simulink model "NBMS_SoC"  (R2026b)
settings: Solver=FixedStepDiscrete  StopTime=25  FixedStep=0.1
undefined symbols (not defined in the file): BMS_BattSoCDerate_E, BMS_BattTempDerate_E, BMS_MODE_E, CAL_15_SOC_WRN_RVL_THRSH, CAL_15_SOC_WRN_THRSH, CAL_DCHRG_END_THRSH, CAL_DOD, CAL_DOD_MAX_THRSH, CAL_DOD_MIN_THRSH, CAL_ENABLE_SOC_WARN_15, CAL_ENABLE_SOC_WARN_20, CAL_GOLDEN_CHARGE, CAL_GOLDEN_DC, CAL_LOW_SOC_RVL_THRSH, CAL_LOW_SOC_THRSH, CAL_NOMINAL_VOLTAGE, CAL_SOC_WRN_RVL_THRSH, CAL_SOC_WRN_THRSH, CAL_SOH_Enable, Charger_Mode_Req_E, DiscIntNeverNeededParam, OBC_E, VDU_MACHINE_STS_E, X_DCIR_CHG, X_DCIR_DISCH, Y_DCIR_CHG, Y_DCIR_DISCH
libraries: simulink x110, simulink_extras x6, sl_discontinuities x3
(part 3 of 3)

== system NBMS_SoC/SOC/VtAvg/Voltage Average/Moving Average10 ==
  note: 2sec Holding the Average
  In : Inport
  EnableCellVoltValid : EnablePort
  20Delay : simulink/Discrete/Tapped Delay  vinit=0.0  samptime=-1  NumDelays=20  DelayOrder=Newest  includeCurrent=off
  Average : Product  Inputs=*/  OutDataTypeStr=fixdt(1,16,0.001,0)
  CountStep : Constant  OutDataTypeStr=uint8
  Counter : Sum  AccumDataTypeStr=uint8  SaturateOnIntegerOverflow=on
  Counterfor20 : Switch  Criteria=u2 > Threshold  Threshold=20  SaturateOnIntegerOverflow=off  InputSameDT=off
  Delayfor1Unit : UnitDelay  SampleTime=-1
  FixdtDataTypeConversion : DataTypeConversion  OutDataTypeStr=fixdt(1,16,0.001,0)  SaturateOnIntegerOverflow=off  RndMeth=Floor
  SumofVoltage : Sum  Inputs=+  OutDataTypeStr=fixdt(1,32,0.001,0)  AccumDataTypeStr=fixdt(1,32,0.001,0)
  TotalCount : Constant  Value=21  OutDataTypeStr=fixdt(1,16,0.001,0)
  TotalSum : Sum  OutDataTypeStr=fixdt(1,32,0.001,0)  AccumDataTypeStr=fixdt(1,32,0.001,0)
  ZeroVt : Constant  Value=0  OutDataTypeStr=fixdt(1,16,0.001,0)
  Out : Outport
  wires:
  CountStep/1 -> Counter/1  "CounterIncrement"
  ZeroVt/1 -> Counterfor20/3  "ZeroVoltage"
  TotalCount/1 -> Average/2  "TotalSample"
  SumofVoltage/1 -> TotalSum/1  "AccumulatedSumof20Vt"
  Counter/1 -> Counterfor20/2, Delayfor1Unit/1  "CounterValue"
  In/1 -> FixdtDataTypeConversion/1  "VoltCell10"
  Delayfor1Unit/1 -> Counter/2  "PreviousValue"
  20Delay/1 -> SumofVoltage/1  "SampleDelayed20"
  FixdtDataTypeConversion/1 -> TotalSum/2, 20Delay/1  "21stVoltage"
  Counterfor20/1 -> Out/1  "AvgVoltofCell10"
  Average/1 -> Counterfor20/1  "AverageVolt"
  TotalSum/1 -> Average/1  "SumofallVolt"

== system NBMS_SoC/SOC/VtAvg/Voltage Average/Moving Average11 ==
  note: 2sec Holding the Average
  In : Inport
  EnableCellVoltValid : EnablePort
  20Delay : simulink/Discrete/Tapped Delay  vinit=0.0  samptime=-1  NumDelays=20  DelayOrder=Newest  includeCurrent=off
  Average : Product  Inputs=*/  OutDataTypeStr=fixdt(1,16,0.001,0)
  CountStep : Constant  OutDataTypeStr=uint8
  Counter : Sum  AccumDataTypeStr=uint8  SaturateOnIntegerOverflow=on
  Counterfor20 : Switch  Criteria=u2 > Threshold  Threshold=20  SaturateOnIntegerOverflow=off  InputSameDT=off
  Delayfor1Unit : UnitDelay  SampleTime=-1
  FixdtDataTypeConversion : DataTypeConversion  OutDataTypeStr=fixdt(1,16,0.001,0)  SaturateOnIntegerOverflow=off  RndMeth=Floor
  SumofVoltage : Sum  Inputs=+  OutDataTypeStr=fixdt(1,32,0.001,0)  AccumDataTypeStr=fixdt(1,32,0.001,0)
  TotalCount : Constant  Value=21  OutDataTypeStr=fixdt(1,16,0.001,0)
  TotalSum : Sum  OutDataTypeStr=fixdt(1,32,0.001,0)  AccumDataTypeStr=fixdt(1,32,0.001,0)
  ZeroVt : Constant  Value=0  OutDataTypeStr=fixdt(1,16,0.001,0)
  Out : Outport
  wires:
  CountStep/1 -> Counter/1  "CounterIncrement"
  ZeroVt/1 -> Counterfor20/3  "ZeroVoltage"
  TotalCount/1 -> Average/2  "TotalSample"
  SumofVoltage/1 -> TotalSum/1  "AccumulatedSumof20Vt"
  Counter/1 -> Counterfor20/2, Delayfor1Unit/1  "CounterValue"
  In/1 -> FixdtDataTypeConversion/1  "VoltCell11"
  Delayfor1Unit/1 -> Counter/2  "PreviousValue"
  20Delay/1 -> SumofVoltage/1  "SampleDelayed20"
  FixdtDataTypeConversion/1 -> TotalSum/2, 20Delay/1  "21stVoltage"
  Counterfor20/1 -> Out/1  "AvgVoltofCell11"
  Average/1 -> Counterfor20/1  "AverageVolt"
  TotalSum/1 -> Average/1  "SumofallVolt"

== system NBMS_SoC/SOC/VtAvg/Voltage Average/Moving Average12 ==
  note: 2sec Holding the Average
  In : Inport
  EnableCellVoltValid : EnablePort
  20Delay : simulink/Discrete/Tapped Delay  vinit=0.0  samptime=-1  NumDelays=20  DelayOrder=Newest  includeCurrent=off
  Average : Product  Inputs=*/  OutDataTypeStr=fixdt(1,16,0.001,0)
  CountStep : Constant  OutDataTypeStr=uint8
  Counter : Sum  AccumDataTypeStr=uint8  SaturateOnIntegerOverflow=on
  Counterfor20 : Switch  Criteria=u2 > Threshold  Threshold=20  SaturateOnIntegerOverflow=off  InputSameDT=off
  Delayfor1Unit : UnitDelay  SampleTime=-1
  FixdtDataTypeConversion : DataTypeConversion  OutDataTypeStr=fixdt(1,16,0.001,0)  SaturateOnIntegerOverflow=off  RndMeth=Floor
  SumofVoltage : Sum  Inputs=+  OutDataTypeStr=fixdt(1,32,0.001,0)  AccumDataTypeStr=fixdt(1,32,0.001,0)
  TotalCount : Constant  Value=21  OutDataTypeStr=fixdt(1,16,0.001,0)
  TotalSum : Sum  OutDataTypeStr=fixdt(1,32,0.001,0)  AccumDataTypeStr=fixdt(1,32,0.001,0)
  ZeroVt : Constant  Value=0  OutDataTypeStr=fixdt(1,16,0.001,0)
  Out : Outport
  wires:
  CountStep/1 -> Counter/1  "CounterIncrement"
  ZeroVt/1 -> Counterfor20/3  "ZeroVoltage"
  TotalCount/1 -> Average/2  "TotalSample"
  SumofVoltage/1 -> TotalSum/1  "AccumulatedSumof20Vt"
  Counter/1 -> Counterfor20/2, Delayfor1Unit/1  "CounterValue"
  In/1 -> FixdtDataTypeConversion/1  "VoltCell12"
  Delayfor1Unit/1 -> Counter/2  "PreviousValue"
  20Delay/1 -> SumofVoltage/1  "SampleDelayed20"
  FixdtDataTypeConversion/1 -> TotalSum/2, 20Delay/1  "21stVoltage"
  Counterfor20/1 -> Out/1  "AvgVoltofCell12"
  Average/1 -> Counterfor20/1  "AverageVolt"
  TotalSum/1 -> Average/1  "SumofallVolt"

== system NBMS_SoC/SOC/VtAvg/Voltage Average/Moving Average13 ==
  note: 2sec Holding the Average
  In : Inport
  EnableCellVoltValid : EnablePort
  20Delay : simulink/Discrete/Tapped Delay  vinit=0.0  samptime=-1  NumDelays=20  DelayOrder=Newest  includeCurrent=off
  Average : Product  Inputs=*/  OutDataTypeStr=fixdt(1,16,0.001,0)
  CountStep : Constant  OutDataTypeStr=uint8
  Counter : Sum  AccumDataTypeStr=uint8  SaturateOnIntegerOverflow=on
  Counterfor20 : Switch  Criteria=u2 > Threshold  Threshold=20  SaturateOnIntegerOverflow=off  InputSameDT=off
  Delayfor1Unit : UnitDelay  SampleTime=-1
  FixdtDataTypeConversion : DataTypeConversion  OutDataTypeStr=fixdt(1,16,0.001,0)  SaturateOnIntegerOverflow=off  RndMeth=Floor
  SumofVoltage : Sum  Inputs=+  OutDataTypeStr=fixdt(1,32,0.001,0)  AccumDataTypeStr=fixdt(1,32,0.001,0)
  TotalCount : Constant  Value=21  OutDataTypeStr=fixdt(1,16,0.001,0)
  TotalSum : Sum  OutDataTypeStr=fixdt(1,32,0.001,0)  AccumDataTypeStr=fixdt(1,32,0.001,0)
  ZeroVt : Constant  Value=0  OutDataTypeStr=fixdt(1,16,0.001,0)
  Out : Outport
  wires:
  CountStep/1 -> Counter/1  "CounterIncrement"
  ZeroVt/1 -> Counterfor20/3  "ZeroVoltage"
  TotalCount/1 -> Average/2  "TotalSample"
  SumofVoltage/1 -> TotalSum/1  "AccumulatedSumof20Vt"
  Counter/1 -> Counterfor20/2, Delayfor1Unit/1  "CounterValue"
  In/1 -> FixdtDataTypeConversion/1  "VoltCell13"
  Delayfor1Unit/1 -> Counter/2  "PreviousValue"
  20Delay/1 -> SumofVoltage/1  "SampleDelayed20"
  FixdtDataTypeConversion/1 -> TotalSum/2, 20Delay/1  "21stVoltage"
  Counterfor20/1 -> Out/1  "AvgVoltofCell13"
  Average/1 -> Counterfor20/1  "AverageVolt"
  TotalSum/1 -> Average/1  "SumofallVolt"

== system NBMS_SoC/SOC/VtAvg/Voltage Average/Moving Average14 ==
  note: 2sec Holding the Average
  In : Inport
  EnableCellVoltValid : EnablePort
  20Delay : simulink/Discrete/Tapped Delay  vinit=0.0  samptime=-1  NumDelays=20  DelayOrder=Newest  includeCurrent=off
  Average : Product  Inputs=*/  OutDataTypeStr=fixdt(1,16,0.001,0)
  CountStep : Constant  OutDataTypeStr=uint8
  Counter : Sum  AccumDataTypeStr=uint8  SaturateOnIntegerOverflow=on
  Counterfor20 : Switch  Criteria=u2 > Threshold  Threshold=20  SaturateOnIntegerOverflow=off  InputSameDT=off
  Delayfor1Unit : UnitDelay  SampleTime=-1
  FixdtDataTypeConversion : DataTypeConversion  OutDataTypeStr=fixdt(1,16,0.001,0)  SaturateOnIntegerOverflow=off  RndMeth=Floor
  SumofVoltage : Sum  Inputs=+  OutDataTypeStr=fixdt(1,32,0.001,0)  AccumDataTypeStr=fixdt(1,32,0.001,0)
  TotalCount : Constant  Value=21  OutDataTypeStr=fixdt(1,16,0.001,0)
  TotalSum : Sum  OutDataTypeStr=fixdt(1,32,0.001,0)  AccumDataTypeStr=fixdt(1,32,0.001,0)
  ZeroVt : Constant  Value=0  OutDataTypeStr=fixdt(1,16,0.001,0)
  Out : Outport
  wires:
  TotalCount/1 -> Average/2  "TotalSample"
  CountStep/1 -> Counter/1  "CounterIncrement"
  Delayfor1Unit/1 -> Counter/2  "PreviousValue"
  In/1 -> FixdtDataTypeConversion/1  "VoltCell14"
  Counter/1 -> Counterfor20/2, Delayfor1Unit/1  "CounterValue"
  SumofVoltage/1 -> TotalSum/1  "AccumulatedSumof20Vt"
  20Delay/1 -> SumofVoltage/1  "SampleDelayed20"
  Average/1 -> Counterfor20/1  "AverageVolt"
  ZeroVt/1 -> Counterfor20/3  "ZeroVoltage"
  TotalSum/1 -> Average/1  "SumofallVolt"
  FixdtDataTypeConversion/1 -> TotalSum/2, 20Delay/1  "21stVoltage"
  Counterfor20/1 -> Out/1  "AvgVoltofCell14"

== system NBMS_SoC/SOC/VtAvg/Voltage Average/Moving Average15 ==
  note: 2sec Holding the Average
  In : Inport
  EnableCellVoltValid : EnablePort
  20Delay : simulink/Discrete/Tapped Delay  vinit=0.0  samptime=-1  NumDelays=20  DelayOrder=Newest  includeCurrent=off
  Average : Product  Inputs=*/  OutDataTypeStr=fixdt(1,16,0.001,0)
  CountStep : Constant  OutDataTypeStr=uint8
  Counter : Sum  AccumDataTypeStr=uint8  SaturateOnIntegerOverflow=on
  Counterfor20 : Switch  Criteria=u2 > Threshold  Threshold=20  SaturateOnIntegerOverflow=off  InputSameDT=off
  Delayfor1Unit : UnitDelay  SampleTime=-1
  FixdtDataTypeConversion : DataTypeConversion  OutDataTypeStr=fixdt(1,16,0.001,0)  SaturateOnIntegerOverflow=off  RndMeth=Floor
  SumofVoltage : Sum  Inputs=+  OutDataTypeStr=fixdt(1,32,0.001,0)  AccumDataTypeStr=fixdt(1,32,0.001,0)
  TotalCount : Constant  Value=21  OutDataTypeStr=fixdt(1,16,0.001,0)
  TotalSum : Sum  OutDataTypeStr=fixdt(1,32,0.001,0)  AccumDataTypeStr=fixdt(1,32,0.001,0)
  ZeroVt : Constant  Value=0  OutDataTypeStr=fixdt(1,16,0.001,0)
  Out : Outport
  wires:
  TotalCount/1 -> Average/2  "TotalSample"
  CountStep/1 -> Counter/1  "CounterIncrement"
  Delayfor1Unit/1 -> Counter/2  "PreviousValue"
  In/1 -> FixdtDataTypeConversion/1  "VoltCell15"
  Counter/1 -> Counterfor20/2, Delayfor1Unit/1  "CounterValue"
  SumofVoltage/1 -> TotalSum/1  "AccumulatedSumof20Vt"
  20Delay/1 -> SumofVoltage/1  "SampleDelayed20"
  Average/1 -> Counterfor20/1  "AverageVolt"
  ZeroVt/1 -> Counterfor20/3  "ZeroVoltage"
  TotalSum/1 -> Average/1  "SumofallVolt"
  FixdtDataTypeConversion/1 -> TotalSum/2, 20Delay/1  "21stVoltage"
  Counterfor20/1 -> Out/1  "AvgVoltofCell15"

== system NBMS_SoC/SOC/VtAvg/Voltage Average/Moving Average16 ==
  note: 2sec Holding the Average
  In : Inport
  EnableCellVoltValid : EnablePort
  20Delay : simulink/Discrete/Tapped Delay  vinit=0.0  samptime=-1  NumDelays=20  DelayOrder=Newest  includeCurrent=off
  Average : Product  Inputs=*/  OutDataTypeStr=fixdt(1,16,0.001,0)
  CountStep : Constant  OutDataTypeStr=uint8
  Counter : Sum  AccumDataTypeStr=uint8  SaturateOnIntegerOverflow=on
  Counterfor20 : Switch  Criteria=u2 > Threshold  Threshold=20  SaturateOnIntegerOverflow=off  InputSameDT=off
  Delayfor1Unit : UnitDelay  SampleTime=-1
  FixdtDataTypeConversion : DataTypeConversion  OutDataTypeStr=fixdt(1,16,0.001,0)  SaturateOnIntegerOverflow=off  RndMeth=Floor
  SumofVoltage : Sum  Inputs=+  OutDataTypeStr=fixdt(1,32,0.001,0)  AccumDataTypeStr=fixdt(1,32,0.001,0)
  TotalCount : Constant  Value=21  OutDataTypeStr=fixdt(1,16,0.001,0)
  TotalSum : Sum  OutDataTypeStr=fixdt(1,32,0.001,0)  AccumDataTypeStr=fixdt(1,32,0.001,0)
  ZeroVt : Constant  Value=0  OutDataTypeStr=fixdt(1,16,0.001,0)
  Out : Outport
  wires:
  TotalCount/1 -> Average/2  "TotalSample"
  CountStep/1 -> Counter/1  "CounterIncrement"
  Delayfor1Unit/1 -> Counter/2  "PreviousValue"
  In/1 -> FixdtDataTypeConversion/1  "VoltCell16"
  Counter/1 -> Counterfor20/2, Delayfor1Unit/1  "CounterValue"
  SumofVoltage/1 -> TotalSum/1  "AccumulatedSumof20Vt"
  20Delay/1 -> SumofVoltage/1  "SampleDelayed20"
  Average/1 -> Counterfor20/1  "AverageVolt"
  ZeroVt/1 -> Counterfor20/3  "ZeroVoltage"
  TotalSum/1 -> Average/1  "SumofallVolt"
  FixdtDataTypeConversion/1 -> TotalSum/2, 20Delay/1  "21stVoltage"
  Counterfor20/1 -> Out/1  "AvgVoltofCell16"

== system NBMS_SoC/SOC/VtAvg/Voltage Average/Moving Average17 ==
  note: 2sec Holding the Average
  In : Inport
  EnableCellVoltValid : EnablePort
  20Delay : simulink/Discrete/Tapped Delay  vinit=0.0  samptime=-1  NumDelays=20  DelayOrder=Newest  includeCurrent=off
  Average : Product  Inputs=*/  OutDataTypeStr=fixdt(1,16,0.001,0)
  CountStep : Constant  OutDataTypeStr=uint8
  Counter : Sum  AccumDataTypeStr=uint8  SaturateOnIntegerOverflow=on
  Counterfor20 : Switch  Criteria=u2 > Threshold  Threshold=20  SaturateOnIntegerOverflow=off  InputSameDT=off
  Delayfor1Unit : UnitDelay  SampleTime=-1
  FixdtDataTypeConversion : DataTypeConversion  OutDataTypeStr=fixdt(1,16,0.001,0)  SaturateOnIntegerOverflow=off  RndMeth=Floor
  SumofVoltage : Sum  Inputs=+  OutDataTypeStr=fixdt(1,32,0.001,0)  AccumDataTypeStr=fixdt(1,32,0.001,0)
  TotalCount : Constant  Value=21  OutDataTypeStr=fixdt(1,16,0.001,0)
  TotalSum : Sum  OutDataTypeStr=fixdt(1,32,0.001,0)  AccumDataTypeStr=fixdt(1,32,0.001,0)
  ZeroVt : Constant  Value=0  OutDataTypeStr=fixdt(1,16,0.001,0)
  Out : Outport
  wires:
  TotalCount/1 -> Average/2  "TotalSample"
  CountStep/1 -> Counter/1  "CounterIncrement"
  Delayfor1Unit/1 -> Counter/2  "PreviousValue"
  In/1 -> FixdtDataTypeConversion/1  "VoltCell17"
  Counter/1 -> Counterfor20/2, Delayfor1Unit/1  "CounterValue"
  SumofVoltage/1 -> TotalSum/1  "AccumulatedSumof20Vt"
  20Delay/1 -> SumofVoltage/1  "SampleDelayed20"
  Average/1 -> Counterfor20/1  "AverageVolt"
  ZeroVt/1 -> Counterfor20/3  "ZeroVoltage"
  TotalSum/1 -> Average/1  "SumofallVolt"
  FixdtDataTypeConversion/1 -> TotalSum/2, 20Delay/1  "21stVoltage"
  Counterfor20/1 -> Out/1  "AvgVoltofCell17"

== system NBMS_SoC/SOC/VtAvg/Voltage Average/Moving Average18 ==
  note: 2sec Holding the Average
  In : Inport
  EnableCellVoltValid : EnablePort
  20Delay : simulink/Discrete/Tapped Delay  vinit=0.0  samptime=-1  NumDelays=20  DelayOrder=Newest  includeCurrent=off
  Average : Product  Inputs=*/  OutDataTypeStr=fixdt(1,16,0.001,0)
  CountStep : Constant  OutDataTypeStr=uint8
  Counter : Sum  AccumDataTypeStr=uint8  SaturateOnIntegerOverflow=on
  Counterfor20 : Switch  Criteria=u2 > Threshold  Threshold=20  SaturateOnIntegerOverflow=off  InputSameDT=off
  Delayfor1Unit : UnitDelay  SampleTime=-1
  FixdtDataTypeConversion : DataTypeConversion  OutDataTypeStr=fixdt(1,16,0.001,0)  SaturateOnIntegerOverflow=off  RndMeth=Floor
  SumofVoltage : Sum  Inputs=+  OutDataTypeStr=fixdt(1,32,0.001,0)  AccumDataTypeStr=fixdt(1,32,0.001,0)
  TotalCount : Constant  Value=21  OutDataTypeStr=fixdt(1,16,0.001,0)
  TotalSum : Sum  OutDataTypeStr=fixdt(1,32,0.001,0)  AccumDataTypeStr=fixdt(1,32,0.001,0)
  ZeroVt : Constant  Value=0  OutDataTypeStr=fixdt(1,16,0.001,0)
  Out : Outport
  wires:
  TotalCount/1 -> Average/2  "TotalSample"
  CountStep/1 -> Counter/1  "CounterIncrement"
  Delayfor1Unit/1 -> Counter/2  "PreviousValue"
  In/1 -> FixdtDataTypeConversion/1  "VoltCell18"
  Counter/1 -> Counterfor20/2, Delayfor1Unit/1  "CounterValue"
  SumofVoltage/1 -> TotalSum/1  "AccumulatedSumof20Vt"
  20Delay/1 -> SumofVoltage/1  "SampleDelayed20"
  Average/1 -> Counterfor20/1  "AverageVolt"
  ZeroVt/1 -> Counterfor20/3  "ZeroVoltage"
  TotalSum/1 -> Average/1  "SumofallVolt"
  FixdtDataTypeConversion/1 -> TotalSum/2, 20Delay/1  "21stVoltage"
  Counterfor20/1 -> Out/1  "AvgVoltofCell18"

== system NBMS_SoC/SOC/VtAvg/Voltage Average/Moving Average19 ==
  note: 2sec Holding the Average
  In : Inport
  EnableCellVoltValid : EnablePort
  20Delay : simulink/Discrete/Tapped Delay  vinit=0.0  samptime=-1  NumDelays=20  DelayOrder=Newest  includeCurrent=off
  Average : Product  Inputs=*/  OutDataTypeStr=fixdt(1,16,0.001,0)
  CountStep : Constant  OutDataTypeStr=uint8
  Counter : Sum  AccumDataTypeStr=uint8  SaturateOnIntegerOverflow=on
  Counterfor20 : Switch  Criteria=u2 > Threshold  Threshold=20  SaturateOnIntegerOverflow=off  InputSameDT=off
  Delayfor1Unit : UnitDelay  SampleTime=-1
  FixdtDataTypeConversion : DataTypeConversion  OutDataTypeStr=fixdt(1,16,0.001,0)  SaturateOnIntegerOverflow=off  RndMeth=Floor
  SumofVoltage : Sum  Inputs=+  OutDataTypeStr=fixdt(1,32,0.001,0)  AccumDataTypeStr=fixdt(1,32,0.001,0)
  TotalCount : Constant  Value=21  OutDataTypeStr=fixdt(1,16,0.001,0)
  TotalSum : Sum  OutDataTypeStr=fixdt(1,32,0.001,0)  AccumDataTypeStr=fixdt(1,32,0.001,0)
  ZeroVt : Constant  Value=0  OutDataTypeStr=fixdt(1,16,0.001,0)
  Out : Outport
  wires:
  TotalCount/1 -> Average/2  "TotalSample"
  CountStep/1 -> Counter/1  "CounterIncrement"
  Delayfor1Unit/1 -> Counter/2  "PreviousValue"
  In/1 -> FixdtDataTypeConversion/1  "VoltCell19"
  Counter/1 -> Counterfor20/2, Delayfor1Unit/1  "CounterValue"
  SumofVoltage/1 -> TotalSum/1  "AccumulatedSumof20Vt"
  20Delay/1 -> SumofVoltage/1  "SampleDelayed20"
  Average/1 -> Counterfor20/1  "AverageVolt"
  ZeroVt/1 -> Counterfor20/3  "ZeroVoltage"
  TotalSum/1 -> Average/1  "SumofallVolt"
  FixdtDataTypeConversion/1 -> TotalSum/2, 20Delay/1  "21stVoltage"
  Counterfor20/1 -> Out/1  "AvgVoltofCell19"

== system NBMS_SoC/SOC/VtAvg/Voltage Average/Moving Average2 ==
  note: 2sec Holding the Average
  In : Inport
  EnableCellVoltValid : EnablePort
  20Delay : simulink/Discrete/Tapped Delay  vinit=0.0  samptime=-1  NumDelays=20  DelayOrder=Newest  includeCurrent=off
  Average : Product  Inputs=*/  OutDataTypeStr=fixdt(1,16,0.001,0)
  CountStep : Constant  OutDataTypeStr=uint8
  Counter : Sum  AccumDataTypeStr=uint8  SaturateOnIntegerOverflow=on
  Counterfor20 : Switch  Criteria=u2 > Threshold  Threshold=20  SaturateOnIntegerOverflow=off  InputSameDT=off
  Delayfor1Unit : UnitDelay  SampleTime=-1
  FixdtDataTypeConversion : DataTypeConversion  OutDataTypeStr=fixdt(1,16,0.001,0)  SaturateOnIntegerOverflow=off  RndMeth=Floor
  SumofVoltage : Sum  Inputs=+  OutDataTypeStr=fixdt(1,32,0.001,0)  AccumDataTypeStr=fixdt(1,32,0.001,0)
  TotalCount : Constant  Value=21  OutDataTypeStr=fixdt(1,16,0.001,0)
  TotalSum : Sum  OutDataTypeStr=fixdt(1,32,0.001,0)  AccumDataTypeStr=fixdt(1,32,0.001,0)
  ZeroVt : Constant  Value=0  OutDataTypeStr=fixdt(1,16,0.001,0)
  Out : Outport
  wires:
  FixdtDataTypeConversion/1 -> TotalSum/2, 20Delay/1  "21stVoltage"
  Counterfor20/1 -> Out/1  "AvgVoltofCell2"
  TotalSum/1 -> Average/1  "SumofallVolt"
  In/1 -> FixdtDataTypeConversion/1  "VoltCell2"
  SumofVoltage/1 -> TotalSum/1  "AccumulatedSumof20Vt"
  CountStep/1 -> Counter/1  "CounterIncrement"
  ZeroVt/1 -> Counterfor20/3  "ZeroVoltage"
  20Delay/1 -> SumofVoltage/1  "SampleDelayed20"
  Delayfor1Unit/1 -> Counter/2  "PreviousValue"
  TotalCount/1 -> Average/2  "TotalSample"
  Counter/1 -> Counterfor20/2, Delayfor1Unit/1  "CounterValue"
  Average/1 -> Counterfor20/1  "AverageVolt"

== system NBMS_SoC/SOC/VtAvg/Voltage Average/Moving Average3 ==
  note: 2sec Holding the Average
  In : Inport
  EnableCellVoltValid : EnablePort
  20Delay : simulink/Discrete/Tapped Delay  vinit=0.0  samptime=-1  NumDelays=20  DelayOrder=Newest  includeCurrent=off
  Average : Product  Inputs=*/  OutDataTypeStr=fixdt(1,16,0.001,0)
  CountStep : Constant  OutDataTypeStr=uint8
  Counter : Sum  AccumDataTypeStr=uint8  SaturateOnIntegerOverflow=on
  Counterfor20 : Switch  Criteria=u2 > Threshold  Threshold=20  SaturateOnIntegerOverflow=off  InputSameDT=off
  Delayfor1Unit : UnitDelay  SampleTime=-1
  FixdtDataTypeConversion : DataTypeConversion  OutDataTypeStr=fixdt(1,16,0.001,0)  SaturateOnIntegerOverflow=off  RndMeth=Floor
  SumofVoltage : Sum  Inputs=+  OutDataTypeStr=fixdt(1,32,0.001,0)  AccumDataTypeStr=fixdt(1,32,0.001,0)
  TotalCount : Constant  Value=21  OutDataTypeStr=fixdt(1,16,0.001,0)
  TotalSum : Sum  OutDataTypeStr=fixdt(1,32,0.001,0)  AccumDataTypeStr=fixdt(1,32,0.001,0)
  ZeroVt : Constant  Value=0  OutDataTypeStr=fixdt(1,16,0.001,0)
  Out : Outport
  wires:
  TotalSum/1 -> Average/1  "SumofallVolt"
  Counterfor20/1 -> Out/1  "AvgVoltofCell3"
  FixdtDataTypeConversion/1 -> TotalSum/2, 20Delay/1  "21stVoltage"
  Average/1 -> Counterfor20/1  "AverageVolt"
  Delayfor1Unit/1 -> Counter/2  "PreviousValue"
  Counter/1 -> Counterfor20/2, Delayfor1Unit/1  "CounterValue"
  20Delay/1 -> SumofVoltage/1  "SampleDelayed20"
  ZeroVt/1 -> Counterfor20/3  "ZeroVoltage"
  CountStep/1 -> Counter/1  "CounterIncrement"
  SumofVoltage/1 -> TotalSum/1  "AccumulatedSumof20Vt"
  TotalCount/1 -> Average/2  "TotalSample"
  In/1 -> FixdtDataTypeConversion/1  "VoltCell3"

== system NBMS_SoC/SOC/VtAvg/Voltage Average/Moving Average4 ==
  note: 2sec Holding the Average
  In : Inport
  EnableCellVoltValid : EnablePort
  20Delay : simulink/Discrete/Tapped Delay  vinit=0.0  samptime=-1  NumDelays=20  DelayOrder=Newest  includeCurrent=off
  Average : Product  Inputs=*/  OutDataTypeStr=fixdt(1,16,0.001,0)
  CountStep : Constant  OutDataTypeStr=uint8
  Counter : Sum  AccumDataTypeStr=uint8  SaturateOnIntegerOverflow=on
  Counterfor20 : Switch  Criteria=u2 > Threshold  Threshold=20  SaturateOnIntegerOverflow=off  InputSameDT=off
  Delayfor1Unit : UnitDelay  SampleTime=-1
  FixdtDataTypeConversion : DataTypeConversion  OutDataTypeStr=fixdt(1,16,0.001,0)  SaturateOnIntegerOverflow=off  RndMeth=Floor
  SumofVoltage : Sum  Inputs=+  OutDataTypeStr=fixdt(1,32,0.001,0)  AccumDataTypeStr=fixdt(1,32,0.001,0)
  TotalCount : Constant  Value=21  OutDataTypeStr=fixdt(1,16,0.001,0)
  TotalSum : Sum  OutDataTypeStr=fixdt(1,32,0.001,0)  AccumDataTypeStr=fixdt(1,32,0.001,0)
  ZeroVt : Constant  Value=0  OutDataTypeStr=fixdt(1,16,0.001,0)
  Out : Outport
  wires:
  CountStep/1 -> Counter/1  "CounterIncrement"
  ZeroVt/1 -> Counterfor20/3  "ZeroVoltage"
  TotalCount/1 -> Average/2  "TotalSample"
  SumofVoltage/1 -> TotalSum/1  "AccumulatedSumof20Vt"
  Counter/1 -> Counterfor20/2, Delayfor1Unit/1  "CounterValue"
  In/1 -> FixdtDataTypeConversion/1  "VoltCell4"
  Delayfor1Unit/1 -> Counter/2  "PreviousValue"
  20Delay/1 -> SumofVoltage/1  "SampleDelayed20"
  FixdtDataTypeConversion/1 -> TotalSum/2, 20Delay/1  "21stVoltage"
  Counterfor20/1 -> Out/1  "AvgVoltofCell4"
  Average/1 -> Counterfor20/1  "AverageVolt"
  TotalSum/1 -> Average/1  "SumofallVolt"

== system NBMS_SoC/SOC/VtAvg/Voltage Average/Moving Average5 ==
  note: 2sec Holding the Average
  In : Inport
  EnableCellVoltValid : EnablePort
  20Delay : simulink/Discrete/Tapped Delay  vinit=0.0  samptime=-1  NumDelays=20  DelayOrder=Newest  includeCurrent=off
  Average : Product  Inputs=*/  OutDataTypeStr=fixdt(1,16,0.001,0)
  CountStep : Constant  OutDataTypeStr=uint8
  Counter : Sum  AccumDataTypeStr=uint8  SaturateOnIntegerOverflow=on
  Counterfor20 : Switch  Criteria=u2 > Threshold  Threshold=20  SaturateOnIntegerOverflow=off  InputSameDT=off
  Delayfor1Unit : UnitDelay  SampleTime=-1
  FixdtDataTypeConversion : DataTypeConversion  OutDataTypeStr=fixdt(1,16,0.001,0)  SaturateOnIntegerOverflow=off  RndMeth=Floor
  SumofVoltage : Sum  Inputs=+  OutDataTypeStr=fixdt(1,32,0.001,0)  AccumDataTypeStr=fixdt(1,32,0.001,0)
  TotalCount : Constant  Value=21  OutDataTypeStr=fixdt(1,16,0.001,0)
  TotalSum : Sum  OutDataTypeStr=fixdt(1,32,0.001,0)  AccumDataTypeStr=fixdt(1,32,0.001,0)
  ZeroVt : Constant  Value=0  OutDataTypeStr=fixdt(1,16,0.001,0)
  Out : Outport
  wires:
  CountStep/1 -> Counter/1  "CounterIncrement"
  ZeroVt/1 -> Counterfor20/3  "ZeroVoltage"
  TotalCount/1 -> Average/2  "TotalSample"
  SumofVoltage/1 -> TotalSum/1  "AccumulatedSumof20Vt"
  Counter/1 -> Counterfor20/2, Delayfor1Unit/1  "CounterValue"
  In/1 -> FixdtDataTypeConversion/1  "VoltCell5"
  Delayfor1Unit/1 -> Counter/2  "PreviousValue"
  20Delay/1 -> SumofVoltage/1  "SampleDelayed20"
  FixdtDataTypeConversion/1 -> TotalSum/2, 20Delay/1  "21stVoltage"
  Counterfor20/1 -> Out/1  "AvgVoltofCell5"
  Average/1 -> Counterfor20/1  "AverageVolt"
  TotalSum/1 -> Average/1  "SumofallVolt"

== system NBMS_SoC/SOC/VtAvg/Voltage Average/Moving Average6 ==
  note: 2sec Holding the Average
  In : Inport
  EnableCellVoltValid : EnablePort
  20Delay : simulink/Discrete/Tapped Delay  vinit=0.0  samptime=-1  NumDelays=20  DelayOrder=Newest  includeCurrent=off
  Average : Product  Inputs=*/  OutDataTypeStr=fixdt(1,16,0.001,0)
  CountStep : Constant  OutDataTypeStr=uint8
  Counter : Sum  AccumDataTypeStr=uint8  SaturateOnIntegerOverflow=on
  Counterfor20 : Switch  Criteria=u2 > Threshold  Threshold=20  SaturateOnIntegerOverflow=off  InputSameDT=off
  Delayfor1Unit : UnitDelay  SampleTime=-1
  FixdtDataTypeConversion : DataTypeConversion  OutDataTypeStr=fixdt(1,16,0.001,0)  SaturateOnIntegerOverflow=off  RndMeth=Floor
  SumofVoltage : Sum  Inputs=+  OutDataTypeStr=fixdt(1,32,0.001,0)  AccumDataTypeStr=fixdt(1,32,0.001,0)
  TotalCount : Constant  Value=21  OutDataTypeStr=fixdt(1,16,0.001,0)
  TotalSum : Sum  OutDataTypeStr=fixdt(1,32,0.001,0)  AccumDataTypeStr=fixdt(1,32,0.001,0)
  ZeroVt : Constant  Value=0  OutDataTypeStr=fixdt(1,16,0.001,0)
  Out : Outport
  wires:
  CountStep/1 -> Counter/1  "CounterIncrement"
  ZeroVt/1 -> Counterfor20/3  "ZeroVoltage"
  TotalCount/1 -> Average/2  "TotalSample"
  SumofVoltage/1 -> TotalSum/1  "AccumulatedSumof20Vt"
  Counter/1 -> Counterfor20/2, Delayfor1Unit/1  "CounterValue"
  In/1 -> FixdtDataTypeConversion/1  "VoltCell6"
  Delayfor1Unit/1 -> Counter/2  "PreviousValue"
  20Delay/1 -> SumofVoltage/1  "SampleDelayed20"
  FixdtDataTypeConversion/1 -> TotalSum/2, 20Delay/1  "21stVoltage"
  Counterfor20/1 -> Out/1  "AvgVoltofCell6"
  Average/1 -> Counterfor20/1  "AverageVolt"
  TotalSum/1 -> Average/1  "SumofallVolt"

== system NBMS_SoC/SOC/VtAvg/Voltage Average/Moving Average7 ==
  note: 2sec Holding the Average
  In : Inport
  EnableCellVoltValid : EnablePort
  20Delay : simulink/Discrete/Tapped Delay  vinit=0.0  samptime=-1  NumDelays=20  DelayOrder=Newest  includeCurrent=off
  Average : Product  Inputs=*/  OutDataTypeStr=fixdt(1,16,0.001,0)
  CountStep : Constant  OutDataTypeStr=uint8
  Counter : Sum  AccumDataTypeStr=uint8  SaturateOnIntegerOverflow=on
  Counterfor20 : Switch  Criteria=u2 > Threshold  Threshold=20  SaturateOnIntegerOverflow=off  InputSameDT=off
  Delayfor1Unit : UnitDelay  SampleTime=-1
  FixdtDataTypeConversion : DataTypeConversion  OutDataTypeStr=fixdt(1,16,0.001,0)  SaturateOnIntegerOverflow=off  RndMeth=Floor
  SumofVoltage : Sum  Inputs=+  OutDataTypeStr=fixdt(1,32,0.001,0)  AccumDataTypeStr=fixdt(1,32,0.001,0)
  TotalCount : Constant  Value=21  OutDataTypeStr=fixdt(1,16,0.001,0)
  TotalSum : Sum  OutDataTypeStr=fixdt(1,32,0.001,0)  AccumDataTypeStr=fixdt(1,32,0.001,0)
  ZeroVt : Constant  Value=0  OutDataTypeStr=fixdt(1,16,0.001,0)
  Out : Outport
  wires:
  CountStep/1 -> Counter/1  "CounterIncrement"
  ZeroVt/1 -> Counterfor20/3  "ZeroVoltage"
  TotalCount/1 -> Average/2  "TotalSample"
  SumofVoltage/1 -> TotalSum/1  "AccumulatedSumof20Vt"
  Counter/1 -> Counterfor20/2, Delayfor1Unit/1  "CounterValue"
  In/1 -> FixdtDataTypeConversion/1  "VoltCell7"
  Delayfor1Unit/1 -> Counter/2  "PreviousValue"
  20Delay/1 -> SumofVoltage/1  "SampleDelayed20"
  FixdtDataTypeConversion/1 -> TotalSum/2, 20Delay/1  "21stVoltage"
  Counterfor20/1 -> Out/1  "AvgVoltofCell7"
  Average/1 -> Counterfor20/1  "AverageVolt"
  TotalSum/1 -> Average/1  "SumofallVolt"

== system NBMS_SoC/SOC/VtAvg/Voltage Average/Moving Average8 ==
  note: 2sec Holding the Average
  In : Inport
  EnableCellVoltValid : EnablePort
  20Delay : simulink/Discrete/Tapped Delay  vinit=0.0  samptime=-1  NumDelays=20  DelayOrder=Newest  includeCurrent=off
  Average : Product  Inputs=*/  OutDataTypeStr=fixdt(1,16,0.001,0)
  CountStep : Constant  OutDataTypeStr=uint8
  Counter : Sum  AccumDataTypeStr=uint8  SaturateOnIntegerOverflow=on
  Counterfor20 : Switch  Criteria=u2 > Threshold  Threshold=20  SaturateOnIntegerOverflow=off  InputSameDT=off
  Delayfor1Unit : UnitDelay  SampleTime=-1
  FixdtDataTypeConversion : DataTypeConversion  OutDataTypeStr=fixdt(1,16,0.001,0)  SaturateOnIntegerOverflow=off  RndMeth=Floor
  SumofVoltage : Sum  Inputs=+  OutDataTypeStr=fixdt(1,32,0.001,0)  AccumDataTypeStr=fixdt(1,32,0.001,0)
  TotalCount : Constant  Value=21  OutDataTypeStr=fixdt(1,16,0.001,0)
  TotalSum : Sum  OutDataTypeStr=fixdt(1,32,0.001,0)  AccumDataTypeStr=fixdt(1,32,0.001,0)
  ZeroVt : Constant  Value=0  OutDataTypeStr=fixdt(1,16,0.001,0)
  Out : Outport
  wires:
  CountStep/1 -> Counter/1  "CounterIncrement"
  ZeroVt/1 -> Counterfor20/3  "ZeroVoltage"
  TotalCount/1 -> Average/2  "TotalSample"
  SumofVoltage/1 -> TotalSum/1  "AccumulatedSumof20Vt"
  Counter/1 -> Counterfor20/2, Delayfor1Unit/1  "CounterValue"
  In/1 -> FixdtDataTypeConversion/1  "VoltCell8"
  Delayfor1Unit/1 -> Counter/2  "PreviousValue"
  20Delay/1 -> SumofVoltage/1  "SampleDelayed20"
  FixdtDataTypeConversion/1 -> TotalSum/2, 20Delay/1  "21stVoltage"
  Counterfor20/1 -> Out/1  "AvgVoltofCell8"
  Average/1 -> Counterfor20/1  "AverageVolt"
  TotalSum/1 -> Average/1  "SumofallVolt"

== system NBMS_SoC/SOC/VtAvg/Voltage Average/Moving Average9 ==
  note: 2sec Holding the Average
  In : Inport
  EnableCellVoltValid : EnablePort
  20Delay : simulink/Discrete/Tapped Delay  vinit=0.0  samptime=-1  NumDelays=20  DelayOrder=Newest  includeCurrent=off
  Average : Product  Inputs=*/  OutDataTypeStr=fixdt(1,16,0.001,0)
  CountStep : Constant  OutDataTypeStr=uint8
  Counter : Sum  AccumDataTypeStr=uint8  SaturateOnIntegerOverflow=on
  Counterfor20 : Switch  Criteria=u2 > Threshold  Threshold=20  SaturateOnIntegerOverflow=off  InputSameDT=off
  Delayfor1Unit : UnitDelay  SampleTime=-1
  FixdtDataTypeConversion : DataTypeConversion  OutDataTypeStr=fixdt(1,16,0.001,0)  SaturateOnIntegerOverflow=off  RndMeth=Floor
  SumofVoltage : Sum  Inputs=+  OutDataTypeStr=fixdt(1,32,0.001,0)  AccumDataTypeStr=fixdt(1,32,0.001,0)
  TotalCount : Constant  Value=21  OutDataTypeStr=fixdt(1,16,0.001,0)
  TotalSum : Sum  OutDataTypeStr=fixdt(1,32,0.001,0)  AccumDataTypeStr=fixdt(1,32,0.001,0)
  ZeroVt : Constant  Value=0  OutDataTypeStr=fixdt(1,16,0.001,0)
  Out : Outport
  wires:
  CountStep/1 -> Counter/1  "CounterIncrement"
  ZeroVt/1 -> Counterfor20/3  "ZeroVoltage"
  TotalCount/1 -> Average/2  "TotalSample"
  SumofVoltage/1 -> TotalSum/1  "AccumulatedSumof20Vt"
  Counter/1 -> Counterfor20/2, Delayfor1Unit/1  "CounterValue"
  In/1 -> FixdtDataTypeConversion/1  "VoltCell9"
  Delayfor1Unit/1 -> Counter/2  "PreviousValue"
  20Delay/1 -> SumofVoltage/1  "SampleDelayed20"
  FixdtDataTypeConversion/1 -> TotalSum/2, 20Delay/1  "21stVoltage"
  Counterfor20/1 -> Out/1  "AvgVoltofCell9"
  Average/1 -> Counterfor20/1  "AverageVolt"
  TotalSum/1 -> Average/1  "SumofallVolt"

== system NBMS_SoC/SOC/VtAvg/Voltage Average/OneSensorVoltFailure ==
  PackVoltage : Inport
  RawVoltage : Inport  Port=2
  Enable : EnablePort  StatesWhenEnabling=reset
  AverageofSensorVoltFail : Subsystem
  VoltDifference : Sum  Inputs=+-
  FailSensorVolt : Outport  OutputWhenDisabled=reset  InitialOutput=5
  FailSensorVoltAvg : Outport  Port=2  OutputWhenDisabled=reset  InitialOutput=5
  wires:
  PackVoltage/1 -> VoltDifference/1  "PackVoltage"
  RawVoltage/1 -> VoltDifference/2  "RawVoltage"
  VoltDifference/1 -> AverageofSensorVoltFail/1(Raw), FailSensorVolt/1  "SensorVoltFail"
  AverageofSensorVoltFail/1(FailSensorVoltAvg) -> FailSensorVoltAvg/1

== system NBMS_SoC/SOC/SOC Estimation/DisplaySOC/FullCharge/LatchFullSoc ==
  SOC_Full : Inport
  Trigger : TriggerPort  VariantControl=(inherit)  PortDimensions=1
  SOC : Outport  InitialOutput=0
  wires:
  SOC_Full/1 -> SOC/1  "LatchedFullSoC"

== system NBMS_SoC/SOC/VtAvg/Voltage Average/OneSensorVoltFailure/AverageofSensorVoltFail ==
  note: 2 sec holding the average
  Raw : Inport
  20Delay : simulink/Discrete/Tapped Delay  vinit=0.0  samptime=-1  NumDelays=20  DelayOrder=Newest  includeCurrent=off
  Average : Product  Inputs=*/  OutDataTypeStr=fixdt(1,16,0.001,0)
  ConstZeroVt : Constant  Value=0  OutDataTypeStr=fixdt(1,16,0.001,0)
  CountStep : Constant  OutDataTypeStr=uint8
  Counter : Sum  AccumDataTypeStr=uint8  SaturateOnIntegerOverflow=on
  Counterfor20 : Switch  Criteria=u2 > Threshold  Threshold=20  SaturateOnIntegerOverflow=off  InputSameDT=off
  FixdtDataTypeConversion : DataTypeConversion  OutDataTypeStr=fixdt(1,16,0.001,0)  SaturateOnIntegerOverflow=off  RndMeth=Floor
  PreviousValue : UnitDelay  SampleTime=-1
  SumofVoltage : Sum  Inputs=+  OutDataTypeStr=fixdt(1,32,0.001,0)  AccumDataTypeStr=fixdt(1,32,0.001,0)
  TotalCount : Constant  Value=21  OutDataTypeStr=fixdt(1,16,0.001,0)
  TotalSum : Sum  OutDataTypeStr=fixdt(1,32,0.001,0)  AccumDataTypeStr=fixdt(1,32,0.001,0)
  FailSensorVoltAvg : Outport  OutputWhenDisabled=reset  InitialOutput=0
  wires:
  TotalCount/1 -> Average/2  "TotalSampleCount"
  20Delay/1 -> SumofVoltage/1  "VltSampleDelayed20"
  SumofVoltage/1 -> TotalSum/1  "AccumulatedSumof20Vt"
  TotalSum/1 -> Average/1  "SumofallVolt"
  Raw/1 -> FixdtDataTypeConversion/1  "RawVoltage"
  Counter/1 -> PreviousValue/1, Counterfor20/2  "CounterValue"
  PreviousValue/1 -> Counter/2  "PreviousValue"
  CountStep/1 -> Counter/1  "CounterIncrement"
  Counterfor20/1 -> FailSensorVoltAvg/1  "AvgSensorVoltFail"
  ConstZeroVt/1 -> Counterfor20/3  "ZeroVt"
  Average/1 -> Counterfor20/1  "AverageVolt"
  FixdtDataTypeConversion/1 -> TotalSum/2, 20Delay/1  "21stVoltage"

== stateflow chart NBMS_SoC/SOC/SOC Estimation/DisplaySOC/FullCharge/StateWaitCondition ==
  state Decision
    en:
    out=0;
    state In
      en:
      count=0;
    state Out
      en:
      count=0;
      du:
      count=count+1;
    (default) -> In
    In -> Out : [prev==0 &&Enable==1]{out=0;}
    Out -> In : [count>=5]{out=1;}
  data: Enable input; out output; prev input; count local

== stateflow chart NBMS_SoC/SOC/VtAvg/Voltage Average/FindMinAvgVolt ==
  state Minimum
    data=max(Array);
    for i=1:20
    if Array(i)~=0
    data=min(data,Array(i));
    end
    end
  (default) -> Minimum
  data: Array input; data output; i local

== stateflow chart NBMS_SoC/SOC/VtAvg/Voltage Average/FindMinVolt ==
  state Minimum
    data=max(Array);
    for i=1:20
    if Array(i)~=0
    data=min(data,Array(i));
    end
    end
  (default) -> Minimum
  data: Array input; data output; i local

== stateflow chart NBMS_SoC/SOC/SOC Estimation/InitialSocManager ==
  state StoreInitialSOC
    InitialSOC=data;
  state IgnOff
  (default) -> StoreInitialSOC
  StoreInitialSOC -> IgnOff : [Reset==false]
  IgnOff -> StoreInitialSOC : [Reset==true]
  data: data input; InitialSOC output; Reset input

== stateflow chart NBMS_SoC/SOC/SOC Estimation/SOC Overriding Handling/SocStateController ==
  state entry
    en,du:
    A=0;
  state entry1
    en,du:
    A=0;
  state entry2
    en,du:
    A=1;
  state entry3
    en,du:
    A=1;
  (default) -> entry
  entry -> entry1 : [D== 1]
  entry3 -> entry : [BMS_sleep == 1]
  entry1 -> entry2 : [C==1]
  entry2 -> entry3 : [D== 1]
  data: A output; C input; D input; BMS_sleep input

== stateflow chart NBMS_SoC/SOC/VtAvg/AverageSoC/SOC_Init_Decision ==
  state SOC_Init
    state Default
      en:
      Init=0;
    state Charge
      en:
      Init=1;
    state Discharge
      en:
      Init=2;
    (default) -> Default
    (junction 10) -> Default
    Discharge -> (junction 10) : [Ign==0]
    Default -> (junction 6) [order 2] : [BMSMODE == BMS_MODE_E.BMS_DISCHARGE||RTC_Wakeup==true||AppIn_SoCLEDSW==true...
        | ||BMSMODE == BMS_MODE_E.BMS_FAULT]
    (junction 6) -> Discharge
    Default -> Charge [order 1] : [BMSMODE == BMS_MODE_E.BMS_CHARGE]
    Charge -> Default : [BMSMODE ~= BMS_MODE_E.BMS_CHARGE]
  data: Init output uint8; Ign input; BMSMODE input; RTC_Wakeup input; AppIn_SoCLEDSW input
